simulink model "sfChemicalTank"  (R2025b)
settings: Solver=VariableStepAuto  StartTime=0.0  StopTime=3000  RelTol=1e-3
model workspace (MAT data in the model file):
  Sig = Simulink.Signal
  Sig.Dimensions = -1
  Sig.DimensionsMode = 'auto'
  Sig.Complexity = 'auto'
  Sig.SampleTime = -1
  Sig.SamplingMode = 'auto'
  Sig.DataType = 'auto'
  drainRate = -20.17
settings Model: Creator=The MathWorks, Inc.  LastModifiedBy=The MathWorks, Inc.
settings RTWCC: GPUComputeCapability=3.5

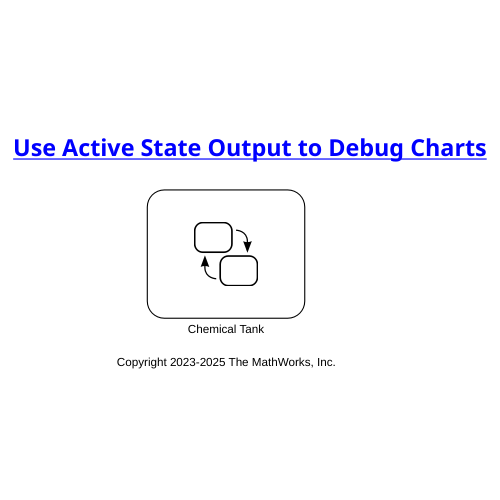
[thumbnail: Simulink's stored preview of the top-level diagram]
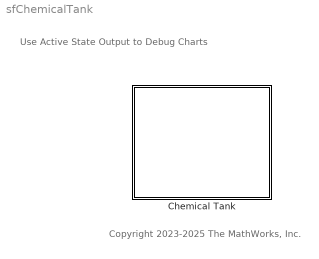
== system sfChemicalTank ==
  note: Copyright 2023-2025 The MathWorks, Inc.
  note: Use Active State Output to Debug Charts
  Chemical Tank : Stateflow chart  TreatAsAtomicUnit=on

== stateflow chart sfChemicalTank/Chemical Tank ==
  state Power_Off
  state Power_On
    state Fill
      during:
      liquid = liquid + pumpRate;
    state Mix
    state Drain
      during:
      liquid = liquid - drainRate;
    state Off
      power = 0;
    state Cool
    (default) -> Fill
    Fill -> Mix : [liquid >= maxVolume]
    Mix -> Drain : after(mixTime, sec)
    Drain -> Cool : [liquid <= minVolume]
    Cool -> Off : after(coolTime, sec)
  (default) -> Power_Off
  Power_Off -> Power_On : [power == 1]
  Power_On -> Power_Off : [power == 0]
  data: power local =1; drainRate local =-1770; pumpRate local =2268; mixTime local =1200; coolTime local =900; liquid local =0; maxVolume local =4000; minVolume local =100
